simulink model "s_c107m32k_vlbi"  (R2018a)
settings: Solver=VariableStepDiscrete  StartTime=0.0  StopTime=(2^15)*10  RelTol=1e-3
undefined symbols (not defined in the file): fft_stages, n_bits_xengs
libraries: xbsIndex_r4 x23049, casper_library_misc x45, xps_library x4, casper_library_scopes x3, simulink x2
(part 5 of 201)

== system s_c107m32k_vlbi/DDC ==
  note: Sync and DV will be inline here
  note: DDS 18.17
  note: Mixer
  note: Filter
  note: Developers note: The coeffs are baked into the block 'UserData' area.
      | The Coeffs are supplied by System Engineering, except implmented at better
      | precision (previous commits the precision was rounded up to 6 decimal places).
      | The coeffs have been added to the User_Data area in the ddc_fir_async
      | blocks (set_param(gcb, 'UserData', coef_107M_6dB_equiripple2) where
      | coef_107M_6dB_equiripple2 was supplied in a .mat file from SE.
      | The coeffs should now 'travel' with the model in full precision.
      | To access: getfield(get_param(gcb, 'UserData'), 'parameters','coeff')
      | is used in the top level model mask.
  sync : Inport
  dvalid : Inport  Port=2
  pol0_data : Inport  Port=3
  osc0 : Inport  Port=4
  pol1_data : Inport  Port=5
  osc1 : Inport  Port=6
  Assert : xbsIndex_r4/Assert  assert_type=on  type_source=Explicitly  gui_display_data_type=Boolean  arith_type=Boolean  n_bits=16  bin_pt=14  preci_type=Single  exp_width=8  frac_width=24  assert_rate=off  rate_source=Explicitly  period=1  output_port=on  block_type=assert
  Concat : xbsIndex_r4/Concat  num_inputs=2  dbl_ovrd=off  block_type=concat
  Concat1 : xbsIndex_r4/Concat  num_inputs=2  dbl_ovrd=off  block_type=concat
  Concat2 : xbsIndex_r4/Concat  num_inputs=2  dbl_ovrd=off  block_type=concat
  Constant : xbsIndex_r4/Constant  const=0  gui_display_data_type=Fixed-point  arith_type=Unsigned  n_bits=8  bin_pt=0  preci_type=Single  exp_width=8  frac_width=24  explicit_period=on  period=1  equ=P=C  opselect=C  inp2=PCIN>>17  opr=+  inp1=P  carry=CIN  dbl_ovrd=off  block_type=constant
  Counter1 : xbsIndex_r4/Counter  Commented=on  cnt_type=Free Running  cnt_to=Inf  operation=Up  start_count=0  cnt_by_val=1  arith_type=Unsigned  n_bits=8  bin_pt=0  load_pin=off  rst=on  en=on  explicit_period=on  period=1  use_behavioral_HDL=off  implementation=DSP48  dbl_ovrd=off  block_type=counter
      settings: block_version=11.4
  Counter2 : xbsIndex_r4/Counter  Commented=on  cnt_type=Free Running  cnt_to=Inf  operation=Up  start_count=0  cnt_by_val=1  arith_type=Unsigned  n_bits=32  bin_pt=0  load_pin=off  rst=on  en=on  explicit_period=on  period=1  use_behavioral_HDL=off  implementation=Fabric  dbl_ovrd=off  block_type=counter
  Counter3 : xbsIndex_r4/Counter  Commented=on  cnt_type=Free Running  cnt_to=Inf  operation=Up  start_count=0  cnt_by_val=1  arith_type=Unsigned  n_bits=8  bin_pt=0  load_pin=off  rst=on  en=on  explicit_period=on  period=1  use_behavioral_HDL=off  implementation=DSP48  dbl_ovrd=off  block_type=counter
      settings: block_version=11.4
  Counter33 : xbsIndex_r4/Counter  Commented=on  cnt_type=Free Running  cnt_to=Inf  operation=Up  start_count=0  cnt_by_val=1  arith_type=Unsigned  n_bits=32  bin_pt=0  load_pin=off  rst=on  en=on  explicit_period=on  period=1  use_behavioral_HDL=off  implementation=Fabric  dbl_ovrd=off  block_type=counter
  Counter4 : xbsIndex_r4/Counter  Commented=on  cnt_type=Free Running  cnt_to=Inf  operation=Up  start_count=0  cnt_by_val=1  arith_type=Unsigned  n_bits=32  bin_pt=0  load_pin=off  rst=on  en=off  explicit_period=on  period=1  use_behavioral_HDL=off  implementation=Fabric  dbl_ovrd=off  block_type=counter
  Counter46 : xbsIndex_r4/Counter  Commented=on  cnt_type=Free Running  cnt_to=Inf  operation=Up  start_count=0  cnt_by_val=1  arith_type=Unsigned  n_bits=32  bin_pt=0  load_pin=off  rst=on  en=off  explicit_period=on  period=1  use_behavioral_HDL=off  implementation=Fabric  dbl_ovrd=off  block_type=counter
  Delay{1..2,4,6..9} (7 alike) : xbsIndex_r4/Delay  rst=off  infoeditControl=Selection of Reset will increase slice count due to use of real FFs and instead of SRLs  en=off  latency=1  reg_retiming=off  dbl_ovrd=off  block_type=delay
      settings: infoedit=Hardware notes: A delay line is a chain, each link of which is an SRL16 or SRL32 followed by a flip-flop.
  Delay3 : xbsIndex_r4/Delay  rst=off  infoeditControl=Selection of Reset will increase slice count due to use of real FFs and instead of SRLs  en=on  latency=1  reg_retiming=off  dbl_ovrd=off  block_type=delay
      settings: infoedit=Hardware notes: A delay line is a chain, each link of which is an SRL16 or SRL32 followed by a flip-flop.
  Delay5 : xbsIndex_r4/Delay  rst=off  infoeditControl=Selection of Reset will increase slice count due to use of real FFs and instead of SRLs  en=on  latency=1  reg_retiming=off  dbl_ovrd=off  block_type=delay
      settings: infoedit=Hardware notes: A delay line is a chain, each link of which is an SRL16 or SRL32 followed by a flip-flop.
  From{2,6,13,16,18,21,33} (7 alike) : From  Commented=on  GotoTag=dec_sync  TagVisibility=global
  From{4,17,22,34} (4 alike) : From  Commented=on  GotoTag=ddc_sync
  From19 : From  Commented=on  GotoTag=dec_d80_0  TagVisibility=global
  From20 : From  Commented=on  GotoTag=cnt_rst  TagVisibility=global
      settings: CloseFcn=tagdialog Close
  From23 : From  Commented=on  GotoTag=ddc_pol0
  From28 : From  Commented=on  GotoTag=cnt_rst  TagVisibility=global
      settings: CloseFcn=tagdialog Close
  From3 : From  Commented=on  GotoTag=dec_dv  TagVisibility=global
  Gateway Out1 : xbsIndex_r4/Gateway Out  inherit_from_input=off  hdl_port=on  rows=1  columns=1  UseAsDAC=off  DACChannel='1'  interface=None  automatic_assignment=on  address_offset=hex2dec('00')  intf_name=''  intf_description=''  timing_constraint=None  locs_specified=off  LOCs={}  io_standard={}  block_type=gatewayout
  Gateway Out2 : xbsIndex_r4/Gateway Out  inherit_from_input=off  hdl_port=on  rows=1  columns=1  UseAsDAC=off  DACChannel='1'  interface=None  automatic_assignment=on  address_offset=hex2dec('00')  intf_name=''  intf_description=''  timing_constraint=None  locs_specified=off  LOCs={}  io_standard={}  block_type=gatewayout
  Inverter : xbsIndex_r4/Inverter  en=off  latency=0  dbl_ovrd=off  block_type=inv
  Logical : xbsIndex_r4/Logical  Commented=on  logical_function=OR  inputs=2  en=off  latency=0  precision=Full  arith_type=Unsigned  n_bits=16  bin_pt=0  align_bp=on  dbl_ovrd=off  block_type=logical
  Logical1 : xbsIndex_r4/Logical  logical_function=AND  inputs=2  en=off  latency=0  precision=Full  arith_type=Unsigned  n_bits=16  bin_pt=0  align_bp=on  dbl_ovrd=off  block_type=logical
  Logical2 : xbsIndex_r4/Logical  logical_function=AND  inputs=2  en=off  latency=0  precision=Full  arith_type=Unsigned  n_bits=16  bin_pt=0  align_bp=on  dbl_ovrd=off  block_type=logical
  Logical29 : xbsIndex_r4/Logical  Commented=on  logical_function=AND  inputs=2  en=off  latency=0  precision=Full  arith_type=Unsigned  n_bits=16  bin_pt=0  align_bp=on  dbl_ovrd=off  block_type=logical
  Logical3 : xbsIndex_r4/Logical  Commented=on  logical_function=AND  inputs=2  en=off  latency=0  precision=Full  arith_type=Unsigned  n_bits=16  bin_pt=0  align_bp=on  dbl_ovrd=off  block_type=logical
  Register : xbsIndex_r4/Register  init=0  rst=off  en=on  dbl_ovrd=off  block_type=register
  Register1 : xbsIndex_r4/Register  init=0  rst=on  en=on  dbl_ovrd=off  block_type=register
  Register2 : xbsIndex_r4/Register  init=0  rst=on  en=on  dbl_ovrd=off  block_type=register
  Register{4..7,24,37,49,62} (8 alike) : xbsIndex_r4/Register  Commented=on  init=0  rst=on  en=on  dbl_ovrd=off  block_type=register
  Register3 : xbsIndex_r4/Register  init=0  rst=off  en=on  dbl_ovrd=off  block_type=register
  Relational : xbsIndex_r4/Relational  mode=a!=b  op_type=Bool  en=off  latency=1  dbl_ovrd=off  block_type=relational
  Relational1 : xbsIndex_r4/Relational  mode=a!=b  op_type=Bool  en=off  latency=1  dbl_ovrd=off  block_type=relational
  Slice1 : xbsIndex_r4/Slice  Commented=on  nbits=32  boolean_output=off  mode=Lower Bit Location + Width  bit1=0  base1=MSB of Input  bit0=0  base0=LSB of Input  dbl_ovrd=off  block_type=slice
  Slice34 : xbsIndex_r4/Slice  Commented=on  nbits=32  boolean_output=off  mode=Lower Bit Location + Width  bit1=0  base1=MSB of Input  bit0=0  base0=LSB of Input  dbl_ovrd=off  block_type=slice
  Terminator : Terminator
  Terminator1 : Terminator
  To Workspace1 : ToWorkspace  VariableName=mult_sync  SaveFormat=Timeseries  SampleTime=-1
  To Workspace2 : ToWorkspace  VariableName=mult_dv  SaveFormat=Timeseries  SampleTime=-1
  bus_convert : Subsystem  AncestorBlock=casper_library_bus/bus_convert  mask(bus_convert){n_bits_in=[29 29 29 29 29 29 29 29], bin_pt_in=26, cmplx=on, n_bits_out=18, bin_pt_out=17, quantization=2, overflow=1, csp_latency=2, of=on, misc=on}
      mask prompts: n_bits_in "input bit widths"; bin_pt_in "input binary points"; cmplx "input complex"; n_bits_out "output bit widths"; bin_pt_out "output binary points"; quantization "quantization strategy (Truncate=0, Round  (unbiased: +/- Inf)=1, Round (unbiased: Even Values)=2)"; overflow "overflow strategy (Wrap=0, Saturate=1, Flag as error=2)"; csp_latency "latency"; of "overflow indication"; misc "misc support"
      mask help: Convert components of busses
      mask init:
      | bus_convert_init(gcb, ...
      |     'n_bits_in', n_bits_in, ...
      |     'bin_pt_in', bin_pt_in, ...
      |     'cmplx', cmplx, ...
      |     'n_bits_out', n_bits_out, ...
      |     'bin_pt_out', bin_pt_out, ...
      |     'quantization', quantization, ...
      |     'overflow', overflow, ...
      |     'csp_latency', csp_latency, ...
      |     'misc', misc, ...
      |     'of', of);
  bus_convert1 : Subsystem  AncestorBlock=casper_library_bus/bus_convert  mask(bus_convert){n_bits_in=[29 29 29 29 29 29 29 29], bin_pt_in=26, cmplx=on, n_bits_out=18, bin_pt_out=17, quantization=2, overflow=1, csp_latency=2, of=on, misc=off}
      mask prompts: n_bits_in "input bit widths"; bin_pt_in "input binary points"; cmplx "input complex"; n_bits_out "output bit widths"; bin_pt_out "output binary points"; quantization "quantization strategy (Truncate=0, Round  (unbiased: +/- Inf)=1, Round (unbiased: Even Values)=2)"; overflow "overflow strategy (Wrap=0, Saturate=1, Flag as error=2)"; csp_latency "latency"; of "overflow indication"; misc "misc support"
      mask help: Convert components of busses
      mask init: same as s_c107m32k_vlbi/DDC/bus_convert
  bus_expand : Subsystem  mask(bus_expand){mode=divisions of equal size, outputNum=2, outputWidth=1, outputBinaryPt=0, outputArithmeticType=2, show_format=off, outputToWorkspace=off, variablePrefix=out, outputToModelAsWell=on}
      mask prompts: outputNum "Number of outputs:"; outputWidth "Output width:"; outputBinaryPt "Output binary point position:"; outputArithmeticType "Output arithmetic type (ufix=0, fix=1, bool=2):"; show_format "Print format string?"; outputToWorkspace "Output to workspace?"; variablePrefix "Variable name prefix:"; outputToModelAsWell "Output to model as well?"
      mask help:
      | Expands a 'bus' made using a bus_create or Xilinx
      | concat block.
      | The input will be divided into the specified number
      | of outputs with the specified arithmetic types.
      | Divisions are made from most significant bit.
      mask init: same as s_c107m32k_vlbi/bus_expand1
      settings: AttributesFormatString=2 outputs
      mask TypeOptions mode: divisions of equal size | divisions of arbitrary size
      mask Callback mode: bus_expand_callback();
      mask Callback outputWidth: bus_expand_callback();
      mask Callback outputToWorkspace: bus_expand_callback();
  bus_expand1 : Subsystem  mask(bus_expand){mode=divisions of equal size, outputNum=16, outputWidth=18, outputBinaryPt=17, outputArithmeticType=1, show_format=off, outputToWorkspace=off, variablePrefix=Sin, outputToModelAsWell=off}
      mask prompts: outputNum "Number of outputs:"; outputWidth "Output width:"; outputBinaryPt "Output binary point position:"; outputArithmeticType "Output arithmetic type (ufix=0, fix=1, bool=2):"; show_format "Print format string?"; outputToWorkspace "Output to workspace?"; variablePrefix "Variable name prefix:"; outputToModelAsWell "Output to model as well?"
      mask help:
      | Expands a 'bus' made using a bus_create or Xilinx
      | concat block.
      | The input will be divided into the specified number
      | of outputs with the specified arithmetic types.
      | Divisions are made from most significant bit.
      mask init: same as s_c107m32k_vlbi/bus_expand1
      settings: AttributesFormatString=16 outputs
      mask TypeOptions mode: divisions of equal size | divisions of arbitrary size
      mask Callback mode: bus_expand_callback();
      mask Callback outputWidth: bus_expand_callback();
      mask Callback outputToWorkspace: bus_expand_callback();
  bus_expand2 : Subsystem  mask(bus_expand){mode=divisions of equal size, outputNum=16, outputWidth=18, outputBinaryPt=17, outputArithmeticType=1, show_format=off, outputToWorkspace=off, variablePrefix=Sin, outputToModelAsWell=off}
      mask prompts: outputNum "Number of outputs:"; outputWidth "Output width:"; outputBinaryPt "Output binary point position:"; outputArithmeticType "Output arithmetic type (ufix=0, fix=1, bool=2):"; show_format "Print format string?"; outputToWorkspace "Output to workspace?"; variablePrefix "Variable name prefix:"; outputToModelAsWell "Output to model as well?"
      mask help:
      | Expands a 'bus' made using a bus_create or Xilinx
      | concat block.
      | The input will be divided into the specified number
      | of outputs with the specified arithmetic types.
      | Divisions are made from most significant bit.
      mask init: same as s_c107m32k_vlbi/bus_expand1
      settings: AttributesFormatString=16 outputs
      mask TypeOptions mode: divisions of equal size | divisions of arbitrary size
      mask Callback mode: bus_expand_callback();
      mask Callback outputWidth: bus_expand_callback();
      mask Callback outputToWorkspace: bus_expand_callback();
  bus_expand5 : Subsystem  mask(bus_expand){mode=divisions of equal size, outputNum=16, outputWidth=18, outputBinaryPt=17, outputArithmeticType=1, show_format=off, outputToWorkspace=off, variablePrefix=Sin, outputToModelAsWell=off}
      mask prompts: outputNum "Number of outputs:"; outputWidth "Output width:"; outputBinaryPt "Output binary point position:"; outputArithmeticType "Output arithmetic type (ufix=0, fix=1, bool=2):"; show_format "Print format string?"; outputToWorkspace "Output to workspace?"; variablePrefix "Variable name prefix:"; outputToModelAsWell "Output to model as well?"
      mask help:
      | Expands a 'bus' made using a bus_create or Xilinx
      | concat block.
      | The input will be divided into the specified number
      | of outputs with the specified arithmetic types.
      | Divisions are made from most significant bit.
      mask init: same as s_c107m32k_vlbi/bus_expand1
      settings: AttributesFormatString=16 outputs
      mask TypeOptions mode: divisions of equal size | divisions of arbitrary size
      mask Callback mode: bus_expand_callback();
      mask Callback outputWidth: bus_expand_callback();
      mask Callback outputToWorkspace: bus_expand_callback();
  bus_expand6 : Subsystem  mask(bus_expand){mode=divisions of equal size, outputNum=16, outputWidth=18, outputBinaryPt=17, outputArithmeticType=1, show_format=off, outputToWorkspace=off, variablePrefix=Sin, outputToModelAsWell=off}
      mask prompts: outputNum "Number of outputs:"; outputWidth "Output width:"; outputBinaryPt "Output binary point position:"; outputArithmeticType "Output arithmetic type (ufix=0, fix=1, bool=2):"; show_format "Print format string?"; outputToWorkspace "Output to workspace?"; variablePrefix "Variable name prefix:"; outputToModelAsWell "Output to model as well?"
      mask help:
      | Expands a 'bus' made using a bus_create or Xilinx
      | concat block.
      | The input will be divided into the specified number
      | of outputs with the specified arithmetic types.
      | Divisions are made from most significant bit.
      mask init: same as s_c107m32k_vlbi/bus_expand1
      settings: AttributesFormatString=16 outputs
      mask TypeOptions mode: divisions of equal size | divisions of arbitrary size
      mask Callback mode: bus_expand_callback();
      mask Callback outputWidth: bus_expand_callback();
      mask Callback outputToWorkspace: bus_expand_callback();
  bus_mult : Subsystem  mask(bus_mult){n_bits_a=[10,10,10,10,10,10,10,10], bin_pt_a=9, type_a=1, cmplx_a=on, n_bits_b=[18,18,18,18,18,18,18,18], bin_pt_b=17, type_b=1, cmplx_b=on, misc=on, floating_point=off, float_type=single, input_vec_a=1, input_vec_b=1, frac_width=19, exp_width=6, n_bits_out=29, bin_pt_out=26, type_out=1, quantization=0, overflow=0, mult_latency=7, add_latency=7, conv_latency=0, max_fanout=1, fan_latency=1, multiplier_implementation=embedded multiplier core, pipeline_cmult_en=off, pipeline_latency=0}
      mask prompts: n_bits_a "a input bit widths"; bin_pt_a "a input binary points"; type_a "a input type (Unsigned=0, Signed=1)"; cmplx_a "a input complex"; n_bits_b "b input bit widths"; bin_pt_b "b input binary points"; type_b "b input type (Unsigned=0, Signed=1)"; cmplx_b "b input complex"; misc "misc support"; floating_point "floating point"; float_type "float type"; input_vec_a "a input vector in bus"; input_vec_b "b input vector in bus"; frac_width "fraction width"; exp_width "exponent width"; n_bits_out "output bit widths"; bin_pt_out "output binary points"; type_out "output type (Unsigned=0, Signed=1)"; quantization "quantization strategy (Truncate=0, Round  (unbiased: +/- Inf)=1)"; overflow "overflow strategy (Wrap=0, Saturate=1, Flag as error=2)"; mult_latency "multiplier latency"; add_latency "adder latency"; conv_latency "convert latency"; max_fanout "limit fanout to ?"; fan_latency "fanout register latency"; multiplier_implementation "multiplier implementation"; pipeline_cmult_en "pipeline complex mult"; pipeline_latency "pipeline latency"
      mask help: Multiply components of two busses
      mask init:
      | bus_mult_init(gcb, ...
      |     'n_bits_a', n_bits_a, ...
      |     'bin_pt_a', bin_pt_a, ...
      |     'type_a', type_a, ...
      |     'cmplx_a', cmplx_a, ...
      |     'n_bits_b', n_bits_b, ...
      |     'bin_pt_b', bin_pt_b, ...
      |     'type_b', type_b, ...
      |     'cmplx_b', cmplx_b, ...
      |     'n_bits_out', n_bits_out, ...
      |     'bin_pt_out', bin_pt_out, ...
      |     'type_out', type_out, ...
      |     'floating_point', floating_point, ...
      |     'float_type', float_type, ...
      |     'exp_width', exp_width, ...
      |     'input_vec_a', input_vec_a, ...
      |     'input_vec_b', input_vec_b, ...
      |     'frac_width', frac_width, ...         
      |     'quantization', quantization, ...
      |     'overflow', overflow, ...
      |     'mult_latency', mult_latency, ...
      |     'add_latency', add_latency, ...
      |     'conv_latency', conv_latency, ...
      |     'max_fanout', max_fanout, ...
      |     'pipeline_cmult_en', pipeline_cmult_en, ...
      |     'pipeline_latency', pipeline_latency, ...
      |     'fan_latency', fan_latency, ...
      |     'multiplier_implementation', multiplier_implementation, ...
      |     'misc', misc);
      mask Callback floating_point:
      | onoff = get_param(gcb, 'floating_point');
      | if strcmp(onoff,'on')
      |     enable_fixpt = 'off'
      |     set_param_state(gcb, 'float_type', 'on')
      | 
      |     set_param_state(gcb, 'input_vec_a', 'on')
      |     set_param_state(gcb, 'input_vec_b', 'on')
      | 
      |     f_type = get_param(gcb, 'float_type')
      |     if strcmp(f_type,'custom')
      |         set_param_state(gcb, 'exp_width', 'on')
      |         set_param_state(gcb, 'frac_width', 'on')
      |     else
      |         set_param_state(gcb, 'exp_width', 'off')
      |         set_param_state(gcb, 'frac_width', 'off')
      |     end
      | 
      | else
      |     enable_fixpt = 'on'
      |     set_param_state(gcb, 'float_type', 'off')
      |     set_param_state(gcb, 'exp_width', 'off')
      |     set_param_state(gcb, 'frac_width', 'off')
      |     set_param_state(gcb, 'input_vec_a', 'off')
      |     set_param_state(gcb, 'input_vec_b', 'off')
      | end
      | 
      | set_param_state(gcb, 'n_bits_a', enable_fixpt)
      | set_param_state(gcb, 'bin_pt_a', enable_fixpt)
      | set_param_state(gcb, 'type_a', enable_fixpt)
      | set_param_state(gcb, 'n_bits_b', enable_fixpt)
      | set_param_state(gcb, 'bin_pt_b', enable_fixpt)
      | set_param_state(gcb, 'type_b', enable_fixpt)
      | 
      | set_param_state(gcb, 'n_bits_out', enable_fixpt)
      | set_param_state(gcb, 'bin_pt_out', enable_fixpt)
      | set_param_state(gcb, 'type_out', enable_fixpt)
      | set_param_state(gcb, 'quantization', enable_fixpt)
      | set_param_state(gcb, 'overflow', enable_fixpt)
      mask TypeOptions float_type: single | custom
      mask Callback float_type:
      | f_type = get_param(gcb, 'float_type')
      | if strcmp(f_type,'custom')
      |     set_param_state(gcb, 'exp_width', 'on')
      |     set_param_state(gcb, 'frac_width', 'on')
      | else
      |     set_param_state(gcb, 'exp_width', 'off')
      |     set_param_state(gcb, 'frac_width', 'off')
      | end
      mask TypeOptions multiplier_implementation: behavioral HDL | standard core | embedded multiplier core
      mask Callback pipeline_cmult_en:
      | pipeline_en = get_param(gcb, 'pipeline_cmult_en');
      | if strcmp(pipeline_en,'on')
      | 
      |     set_param_state(gcb, 'pipeline_latency', 'on')
      | else
      |     set_param_state(gcb, 'pipeline_latency', 'off')
      | end
  bus_mult1 : Subsystem  mask(bus_mult){n_bits_a=[10,10,10,10,10,10,10,10], bin_pt_a=9, type_a=1, cmplx_a=on, n_bits_b=[18,18,18,18,18,18,18,18], bin_pt_b=17, type_b=1, cmplx_b=on, misc=off, floating_point=off, float_type=single, input_vec_a=1, input_vec_b=1, frac_width=19, exp_width=6, n_bits_out=29, bin_pt_out=26, type_out=1, quantization=0, overflow=0, mult_latency=7, add_latency=7, conv_latency=0, max_fanout=1, fan_latency=1, multiplier_implementation=embedded multiplier core, pipeline_cmult_en=off, pipeline_latency=0}
      mask prompts: n_bits_a "a input bit widths"; bin_pt_a "a input binary points"; type_a "a input type (Unsigned=0, Signed=1)"; cmplx_a "a input complex"; n_bits_b "b input bit widths"; bin_pt_b "b input binary points"; type_b "b input type (Unsigned=0, Signed=1)"; cmplx_b "b input complex"; misc "misc support"; floating_point "floating point"; float_type "float type"; input_vec_a "a input vector in bus"; input_vec_b "b input vector in bus"; frac_width "fraction width"; exp_width "exponent width"; n_bits_out "output bit widths"; bin_pt_out "output binary points"; type_out "output type (Unsigned=0, Signed=1)"; quantization "quantization strategy (Truncate=0, Round  (unbiased: +/- Inf)=1)"; overflow "overflow strategy (Wrap=0, Saturate=1, Flag as error=2)"; mult_latency "multiplier latency"; add_latency "adder latency"; conv_latency "convert latency"; max_fanout "limit fanout to ?"; fan_latency "fanout register latency"; multiplier_implementation "multiplier implementation"; pipeline_cmult_en "pipeline complex mult"; pipeline_latency "pipeline latency"
      mask help: Multiply components of two busses
      mask init: same as s_c107m32k_vlbi/DDC/bus_mult
      mask Callback floating_point:
      | onoff = get_param(gcb, 'floating_point');
      | if strcmp(onoff,'on')
      |     enable_fixpt = 'off'
      |     set_param_state(gcb, 'float_type', 'on')
      | 
      |     set_param_state(gcb, 'input_vec_a', 'on')
      |     set_param_state(gcb, 'input_vec_b', 'on')
      | 
      |     f_type = get_param(gcb, 'float_type')
      |     if strcmp(f_type,'custom')
      |         set_param_state(gcb, 'exp_width', 'on')
      |         set_param_state(gcb, 'frac_width', 'on')
      |     else
      |         set_param_state(gcb, 'exp_width', 'off')
      |         set_param_state(gcb, 'frac_width', 'off')
      |     end
      | 
      | else
      |     enable_fixpt = 'on'
      |     set_param_state(gcb, 'float_type', 'off')
      |     set_param_state(gcb, 'exp_width', 'off')
      |     set_param_state(gcb, 'frac_width', 'off')
      |     set_param_state(gcb, 'input_vec_a', 'off')
      |     set_param_state(gcb, 'input_vec_b', 'off')
      | end
      | 
      | set_param_state(gcb, 'n_bits_a', enable_fixpt)
      | set_param_state(gcb, 'bin_pt_a', enable_fixpt)
      | set_param_state(gcb, 'type_a', enable_fixpt)
      | set_param_state(gcb, 'n_bits_b', enable_fixpt)
      | set_param_state(gcb, 'bin_pt_b', enable_fixpt)
      | set_param_state(gcb, 'type_b', enable_fixpt)
      | 
      | set_param_state(gcb, 'n_bits_out', enable_fixpt)
      | set_param_state(gcb, 'bin_pt_out', enable_fixpt)
      | set_param_state(gcb, 'type_out', enable_fixpt)
      | set_param_state(gcb, 'quantization', enable_fixpt)
      | set_param_state(gcb, 'overflow', enable_fixpt)
      mask TypeOptions float_type: single | custom
      mask Callback float_type:
      | f_type = get_param(gcb, 'float_type')
      | if strcmp(f_type,'custom')
      |     set_param_state(gcb, 'exp_width', 'on')
      |     set_param_state(gcb, 'frac_width', 'on')
      | else
      |     set_param_state(gcb, 'exp_width', 'off')
      |     set_param_state(gcb, 'frac_width', 'off')
      | end
      mask TypeOptions multiplier_implementation: behavioral HDL | standard core | embedded multiplier core
      mask Callback pipeline_cmult_en:
      | pipeline_en = get_param(gcb, 'pipeline_cmult_en');
      | if strcmp(pipeline_en,'on')
      | 
      |     set_param_state(gcb, 'pipeline_latency', 'on')
      | else
      |     set_param_state(gcb, 'pipeline_latency', 'off')
      | end
  convert_of : Subsystem  Commented=on  AncestorBlock=casper_library_misc/convert_of  mask(convert_of){bit_width_i=44, binary_point_i=34, bit_width_o=18, binary_point_o=17, latency=2, overflow=Saturate, quantization=Round  (unbiased: +/- Inf)}
      mask prompts: bit_width_i "Bit Width In"; binary_point_i "Binary Point In"; bit_width_o "Bit Width Out"; binary_point_o "Binary Point Out"; overflow "Overflow Behaviour"; quantization "Quantization Behaviour"
      mask help:
      | Converts from one 2's complement bit-width
      | and/or binary point position to another.
      | Includes underflow/overflow indicator.
      mask init:
      | convert_of_init(gcb, ...
      |     'bit_width_i', bit_width_i, ...
      |     'binary_point_i', binary_point_i, ...
      |     'bit_width_o', bit_width_o, ...
      |     'binary_point_o', binary_point_o, ...
      |     'latency', latency, ...
      |     'overflow', overflow, ...
      |     'quantization', quantization);
      settings: AttributesFormatString=[44,34]->[18,17]
      mask TypeOptions overflow: Wrap | Saturate | Error
      mask TypeOptions quantization: Truncate | Round  (unbiased: +/- Inf) | Round  (unbiased: even values)
  convert_of1 : Subsystem  Commented=on  AncestorBlock=casper_library_misc/convert_of  mask(convert_of){bit_width_i=44, binary_point_i=34, bit_width_o=18, binary_point_o=17, latency=2, overflow=Saturate, quantization=Round  (unbiased: +/- Inf)}
      mask prompts: bit_width_i "Bit Width In"; binary_point_i "Binary Point In"; bit_width_o "Bit Width Out"; binary_point_o "Binary Point Out"; overflow "Overflow Behaviour"; quantization "Quantization Behaviour"
      mask help:
      | Converts from one 2's complement bit-width
      | and/or binary point position to another.
      | Includes underflow/overflow indicator.
      mask init: same as s_c107m32k_vlbi/DDC/convert_of
      settings: AttributesFormatString=[44,34]->[18,17]
      mask TypeOptions overflow: Wrap | Saturate | Error
      mask TypeOptions quantization: Truncate | Round  (unbiased: +/- Inf) | Round  (unbiased: even values)
  ddc_in_sync_cnt : Subsystem  Tag=xps:sw_reg  Commented=on  AncestorBlock=xps_library/Memory/software_register  mask(swreg){io_dir=To Processor, io_delay=0, init_val=0, sample_period=1, names=reg, bitwidths=8, bin_pts=0, arith_types=0, sim_port=off, show_format=on}
      mask prompts: io_dir "I/O direction"; io_delay "I/O delay"; init_val "Initial Value"; sample_period "Sample period"; names "Bitfield names [msb...lsb]"; bitwidths "Bitfield widths"; bin_pts "Bitfield binary pts"; arith_types "Bitfield types, ufix=0, fix=1, bool=2"; sim_port "Provide sim input/output?"; show_format "Print format string?"
      mask help: A 32-bit software-accessible register. Can be divided into bitfields of varying widths and types using the fields in the block mask.
      mask init:
      | swreg_init(gcb)
      settings: AttributesFormatString=1output:uf8.0 = 8 bits
      mask TypeOptions io_dir: To Processor | From Processor
      mask Callback io_dir:
      | mask_enables = get_param(gcb, 'MaskEnables');
      | mask_names = get_param(gcb, 'MaskNames');
      | if strcmp(get_param(gcb, 'io_dir'), 'To Processor'),
      |     mask_enables{ismember(mask_names, 'sample_period')} = 'off';
      | else
      |     mask_enables{ismember(mask_names, 'sample_period')} = 'on';
      | end
      | set_param(gcb, 'MaskEnables', mask_enables);
      mask DialogControl ParameterTabVar0 Prompt: Setup
  ddc_out_sync_cnt : Subsystem  Tag=xps:sw_reg  Commented=on  AncestorBlock=xps_library/Memory/software_register  mask(swreg){io_dir=To Processor, io_delay=0, init_val=0, sample_period=1, names=reg, bitwidths=8, bin_pts=0, arith_types=0, sim_port=off, show_format=on}
      mask prompts: io_dir "I/O direction"; io_delay "I/O delay"; init_val "Initial Value"; sample_period "Sample period"; names "Bitfield names [msb...lsb]"; bitwidths "Bitfield widths"; bin_pts "Bitfield binary pts"; arith_types "Bitfield types, ufix=0, fix=1, bool=2"; sim_port "Provide sim input/output?"; show_format "Print format string?"
      mask help: A 32-bit software-accessible register. Can be divided into bitfields of varying widths and types using the fields in the block mask.
      mask init:
      | swreg_init(gcb)
      settings: AttributesFormatString=1output:uf8.0 = 8 bits
      mask TypeOptions io_dir: To Processor | From Processor
      mask Callback io_dir:
      | mask_enables = get_param(gcb, 'MaskEnables');
      | mask_names = get_param(gcb, 'MaskNames');
      | if strcmp(get_param(gcb, 'io_dir'), 'To Processor'),
      |     mask_enables{ismember(mask_names, 'sample_period')} = 'off';
      | else
      |     mask_enables{ismember(mask_names, 'sample_period')} = 'on';
      | end
      | set_param(gcb, 'MaskEnables', mask_enables);
      mask DialogControl ParameterTabVar0 Prompt: Setup
  dec_fir_async : Subsystem  Tag=casper:dec_fir_async  AncestorBlock=casper_library_downconverter/dec_fir_async  mask(dec_fir_async){n_inputs=16, coeff=getfield(get_param(gcb, 'UserData'), 'parameters','coeff'), output_width=18, output_bp=17, quantization=Round  (unbiased: Even Values), add_latency=7, mult_latency=7, conv_latency=7, coeff_bit_width=18, coeff_bin_pt=17, lshift=0, absorb_adders=on, adder_imp=DSP48, async=on, bus_input=off, input_width=0, input_bp=0, input_type=Signed}
      mask prompts: n_inputs "Number of Parallel Streams"; coeff "Coefficients"; output_width "Output bitwidth"; output_bp "Output binary point"; quantization "Quantization Behavior"; add_latency "Add Latency"; mult_latency "Mult Latency"; conv_latency "Convert latency"; coeff_bit_width "Coefficient bitwidth"; coeff_bin_pt "Coefficient binary point"; lshift "Post adder-tree shift"; absorb_adders "Absorb adders into DSP slices"; adder_imp "Adder implementation"; async "Asynchronous ops"; bus_input "Bus input"; input_width "Input bitwidth"; input_bp "Input binary point"; input_type "Input datatype"
      mask help: FIR filter which can handle multiple time samples in parallel and decimates down to 1 time sample. If coefficients are symmetric, will automatically fold before multiplying.
      mask init:
      | dec_fir_async_init(gcb);
      settings: AttributesFormatString=|
      | 256 taps
      | 18_17 r/i
      mask TypeOptions quantization: Truncate | Round  (unbiased: +/- Inf) | Round  (unbiased: Even Values)
      mask TypeOptions adder_imp: Behavioral | Fabric | DSP48
      mask Callback bus_input:
      | onoff = get_param(gcb, 'bus_input');
      | set_param_state(gcb, 'input_width', onoff)
      | set_param_state(gcb, 'input_bp', onoff)
      | set_param_state(gcb, 'input_type', onoff)
      mask TypeOptions input_type: Signed | Unsigned
  dec_fir_async2 : Subsystem  Tag=casper:dec_fir_async  AncestorBlock=casper_library_downconverter/dec_fir_async  mask(dec_fir_async){n_inputs=16, coeff=getfield(get_param(gcb, 'UserData'), 'parameters','coeff'), output_width=18, output_bp=17, quantization=Round  (unbiased: Even Values), add_latency=7, mult_latency=7, conv_latency=7, coeff_bit_width=18, coeff_bin_pt=17, lshift=0, absorb_adders=on, adder_imp=DSP48, async=on, bus_input=off, input_width=0, input_bp=0, input_type=Signed}
      mask prompts: n_inputs "Number of Parallel Streams"; coeff "Coefficients"; output_width "Output bitwidth"; output_bp "Output binary point"; quantization "Quantization Behavior"; add_latency "Add Latency"; mult_latency "Mult Latency"; conv_latency "Convert latency"; coeff_bit_width "Coefficient bitwidth"; coeff_bin_pt "Coefficient binary point"; lshift "Post adder-tree shift"; absorb_adders "Absorb adders into DSP slices"; adder_imp "Adder implementation"; async "Asynchronous ops"; bus_input "Bus input"; input_width "Input bitwidth"; input_bp "Input binary point"; input_type "Input datatype"
      mask help: FIR filter which can handle multiple time samples in parallel and decimates down to 1 time sample. If coefficients are symmetric, will automatically fold before multiplying.
      mask init:
      | dec_fir_async_init(gcb);
      settings: AttributesFormatString=|
      | 256 taps
      | 18_17 r/i
      mask TypeOptions quantization: Truncate | Round  (unbiased: +/- Inf) | Round  (unbiased: Even Values)
      mask TypeOptions adder_imp: Behavioral | Fabric | DSP48
      mask Callback bus_input:
      | onoff = get_param(gcb, 'bus_input');
      | set_param_state(gcb, 'input_width', onoff)
      | set_param_state(gcb, 'input_bp', onoff)
      | set_param_state(gcb, 'input_type', onoff)
      mask TypeOptions input_type: Signed | Unsigned
  edge_detect1 : Subsystem  Commented=on  mask(edge_detect){edge=Rising, polarity=Active High, x_in=[0 0.08 0.08 0.16 0.16 0.24 0.24 0.32 0.32 0.4], y_in=[-1 -1  1  1  1  1  1  1  1  1], x_out=[0.6 0.68 0.68 0.76 0.76 0.84 0.84 0.92 0.92 1], y_out=[-1 -1  1  1 -1 -1 -1 -1 -1 -1]}
      mask prompts: edge "Edge Type"; polarity "Output Polarity"; x_in "Input X Positions"; y_in "Input Y Positions"; x_out "Output X Positions"; y_out "Output Y Positions"
      mask help: Output is active for one-cycle after each edge of the specified type (i.e. rising, falling or both).
      mask init: same as s_c107m32k_vlbi/edge_detect1
      settings: AttributesFormatString=|
      | rising edges
      | active high
      mask Help: Output is active for one-cycle after each edge of the specified type (i.e. rising, falling, or both).  Latency is zero.
      mask TypeOptions edge: Rising | Falling | Both
      mask TypeOptions polarity: Active High | Active Low
      mask Display:
      | plot(x_in_num,0.5+y_in_num*0.2);
      | plot(x_out_num,0.5+y_out_num*0.2);
  edge_detect16 : Subsystem  Commented=on  mask(edge_detect){edge=Rising, polarity=Active High, x_in=[0 0.08 0.08 0.16 0.16 0.24 0.24 0.32 0.32 0.4], y_in=[-1 -1  1  1  1  1  1  1  1  1], x_out=[0.6 0.68 0.68 0.76 0.76 0.84 0.84 0.92 0.92 1], y_out=[-1 -1  1  1 -1 -1 -1 -1 -1 -1]}
      mask prompts: edge "Edge Type"; polarity "Output Polarity"; x_in "Input X Positions"; y_in "Input Y Positions"; x_out "Output X Positions"; y_out "Output Y Positions"
      mask help: Output is active for one-cycle after each edge of the specified type (i.e. rising, falling or both).
      mask init: same as s_c107m32k_vlbi/edge_detect1
      settings: AttributesFormatString=|
      | rising edges
      | active high
      mask Help: Output is active for one-cycle after each edge of the specified type (i.e. rising, falling, or both).  Latency is zero.
      mask TypeOptions edge: Rising | Falling | Both
      mask TypeOptions polarity: Active High | Active Low
      mask Display:
      | plot(x_in_num,0.5+y_in_num*0.2);
      | plot(x_out_num,0.5+y_out_num*0.2);
  edge_detect2 : Subsystem  Commented=on  mask(edge_detect){edge=Rising, polarity=Active High, x_in=[0 0.08 0.08 0.16 0.16 0.24 0.24 0.32 0.32 0.4], y_in=[-1 -1  1  1  1  1  1  1  1  1], x_out=[0.6 0.68 0.68 0.76 0.76 0.84 0.84 0.92 0.92 1], y_out=[-1 -1  1  1 -1 -1 -1 -1 -1 -1]}
      mask prompts: edge "Edge Type"; polarity "Output Polarity"; x_in "Input X Positions"; y_in "Input Y Positions"; x_out "Output X Positions"; y_out "Output Y Positions"
      mask help: Output is active for one-cycle after each edge of the specified type (i.e. rising, falling or both).
      mask init: same as s_c107m32k_vlbi/edge_detect1
      settings: AttributesFormatString=|
      | rising edges
      | active high
      mask Help: Output is active for one-cycle after each edge of the specified type (i.e. rising, falling, or both).  Latency is zero.
      mask TypeOptions edge: Rising | Falling | Both
      mask TypeOptions polarity: Active High | Active Low
      mask Display:
      | plot(x_in_num,0.5+y_in_num*0.2);
      | plot(x_out_num,0.5+y_out_num*0.2);
  edge_detect29 : Subsystem  Commented=on  mask(edge_detect){edge=Rising, polarity=Active High, x_in=[0 0.08 0.08 0.16 0.16 0.24 0.24 0.32 0.32 0.4], y_in=[-1 -1  1  1  1  1  1  1  1  1], x_out=[0.6 0.68 0.68 0.76 0.76 0.84 0.84 0.92 0.92 1], y_out=[-1 -1  1  1 -1 -1 -1 -1 -1 -1]}
      mask prompts: edge "Edge Type"; polarity "Output Polarity"; x_in "Input X Positions"; y_in "Input Y Positions"; x_out "Output X Positions"; y_out "Output Y Positions"
      mask help: Output is active for one-cycle after each edge of the specified type (i.e. rising, falling or both).
      mask init: same as s_c107m32k_vlbi/edge_detect1
      settings: AttributesFormatString=|
      | rising edges
      | active high
      mask Help: Output is active for one-cycle after each edge of the specified type (i.e. rising, falling, or both).  Latency is zero.
      mask TypeOptions edge: Rising | Falling | Both
      mask TypeOptions polarity: Active High | Active Low
      mask Display:
      | plot(x_in_num,0.5+y_in_num*0.2);
      | plot(x_out_num,0.5+y_out_num*0.2);
  edge_detect3 : Subsystem  Commented=on  mask(edge_detect){edge=Falling, polarity=Active High, x_in=[0 0.08 0.08 0.16 0.16 0.24 0.24 0.32 0.32 0.4], y_in=[-1 -1  1  1  1  1  1  1  1  1], x_out=[0.6 0.68 0.68 0.76 0.76 0.84 0.84 0.92 0.92 1], y_out=[-1 -1  1  1 -1 -1 -1 -1 -1 -1]}
      mask prompts: edge "Edge Type"; polarity "Output Polarity"; x_in "Input X Positions"; y_in "Input Y Positions"; x_out "Output X Positions"; y_out "Output Y Positions"
      mask help: Output is active for one-cycle after each edge of the specified type (i.e. rising, falling or both).
      mask init: same as s_c107m32k_vlbi/edge_detect1
      settings: AttributesFormatString=|
      | falling edges
      | active high
      mask Help: Output is active for one-cycle after each edge of the specified type (i.e. rising, falling, or both).  Latency is zero.
      mask TypeOptions edge: Rising | Falling | Both
      mask TypeOptions polarity: Active High | Active Low
      mask Display:
      | plot(x_in_num,0.5+y_in_num*0.2);
      | plot(x_out_num,0.5+y_out_num*0.2);
  edge_detect40 : Subsystem  Commented=on  mask(edge_detect){edge=Rising, polarity=Active High, x_in=[0 0.08 0.08 0.16 0.16 0.24 0.24 0.32 0.32 0.4], y_in=[-1 -1  1  1  1  1  1  1  1  1], x_out=[0.6 0.68 0.68 0.76 0.76 0.84 0.84 0.92 0.92 1], y_out=[-1 -1  1  1 -1 -1 -1 -1 -1 -1]}
      mask prompts: edge "Edge Type"; polarity "Output Polarity"; x_in "Input X Positions"; y_in "Input Y Positions"; x_out "Output X Positions"; y_out "Output Y Positions"
      mask help: Output is active for one-cycle after each edge of the specified type (i.e. rising, falling or both).
      mask init: same as s_c107m32k_vlbi/edge_detect1
      settings: AttributesFormatString=|
      | rising edges
      | active high
      mask Help: Output is active for one-cycle after each edge of the specified type (i.e. rising, falling, or both).  Latency is zero.
      mask TypeOptions edge: Rising | Falling | Both
      mask TypeOptions polarity: Active High | Active Low
      mask Display:
      | plot(x_in_num,0.5+y_in_num*0.2);
      | plot(x_out_num,0.5+y_out_num*0.2);
  edge_detect51 : Subsystem  Commented=on  mask(edge_detect){edge=Falling, polarity=Active High, x_in=[0 0.08 0.08 0.16 0.16 0.24 0.24 0.32 0.32 0.4], y_in=[-1 -1  1  1  1  1  1  1  1  1], x_out=[0.6 0.68 0.68 0.76 0.76 0.84 0.84 0.92 0.92 1], y_out=[-1 -1  1  1 -1 -1 -1 -1 -1 -1]}
      mask prompts: edge "Edge Type"; polarity "Output Polarity"; x_in "Input X Positions"; y_in "Input Y Positions"; x_out "Output X Positions"; y_out "Output Y Positions"
      mask help: Output is active for one-cycle after each edge of the specified type (i.e. rising, falling or both).
      mask init: same as s_c107m32k_vlbi/edge_detect1
      settings: AttributesFormatString=|
      | falling edges
      | active high
      mask Help: Output is active for one-cycle after each edge of the specified type (i.e. rising, falling, or both).  Latency is zero.
      mask TypeOptions edge: Rising | Falling | Both
      mask TypeOptions polarity: Active High | Active Low
      mask Display:
      | plot(x_in_num,0.5+y_in_num*0.2);
      | plot(x_out_num,0.5+y_out_num*0.2);
  pipeline21 : Subsystem  Commented=on  AncestorBlock=casper_library_delays/pipeline  mask(pipeline){latency=2}
      mask help:
      | An explicitly laid-out delay line to avoid mapping to SRL16s
      | for use in pipelining to help achieve timing closure.
      mask init:
      | pipeline_init(gcb,'latency',latency);
      settings: AttributesFormatString=Latency = %<latency>
      mask Display:
      | port_label('input', 1, 'd');
      | port_label('output', 1, 'q');
      | disp(['Z^-', num2str(latency)]);
  pipeline22 : Subsystem  Commented=on  AncestorBlock=casper_library_delays/pipeline  mask(pipeline){latency=2}
      mask help:
      | An explicitly laid-out delay line to avoid mapping to SRL16s
      | for use in pipelining to help achieve timing closure.
      mask init:
      | pipeline_init(gcb,'latency',latency);
      settings: AttributesFormatString=Latency = %<latency>
      mask Display:
      | port_label('input', 1, 'd');
      | port_label('output', 1, 'q');
      | disp(['Z^-', num2str(latency)]);
  pipeline39 : Subsystem  Commented=on  AncestorBlock=casper_library_delays/pipeline  mask(pipeline){latency=2}
      mask help:
      | An explicitly laid-out delay line to avoid mapping to SRL16s
      | for use in pipelining to help achieve timing closure.
      mask init:
      | pipeline_init(gcb,'latency',latency);
      settings: AttributesFormatString=Latency = %<latency>
      mask Display:
      | port_label('input', 1, 'd');
      | port_label('output', 1, 'q');
      | disp(['Z^-', num2str(latency)]);
  pipeline40 : Subsystem  Commented=on  AncestorBlock=casper_library_delays/pipeline  mask(pipeline){latency=2}
      mask help:
      | An explicitly laid-out delay line to avoid mapping to SRL16s
      | for use in pipelining to help achieve timing closure.
      mask init:
      | pipeline_init(gcb,'latency',latency);
      settings: AttributesFormatString=Latency = %<latency>
      mask Display:
      | port_label('input', 1, 'd');
      | port_label('output', 1, 'q');
      | disp(['Z^-', num2str(latency)]);
  ri_to_c1 : casper_library_misc/ri_to_c  Commented=on
      settings: SourceProductName=CASPER DSP Blockset
  sync_lat_decfir : Subsystem  Tag=xps:sw_reg  Commented=on  AncestorBlock=xps_library/Memory/software_register  mask(swreg){io_dir=To Processor, io_delay=0, init_val=0, sample_period=1, names=count, bitwidths=32, bin_pts=0, arith_types=0, sim_port=off, show_format=on}
      mask prompts: io_dir "I/O direction"; io_delay "I/O delay"; init_val "Initial Value"; sample_period "Sample period"; names "Bitfield names [msb...lsb]"; bitwidths "Bitfield widths"; bin_pts "Bitfield binary pts"; arith_types "Bitfield types, ufix=0, fix=1, bool=2"; sim_port "Provide sim input/output?"; show_format "Print format string?"
      mask help: A 32-bit software-accessible register. Can be divided into bitfields of varying widths and types using the fields in the block mask.
      mask init:
      | swreg_init(gcb)
      settings: AttributesFormatString=1output:uf32.0 = 32 bits
      mask TypeOptions io_dir: To Processor | From Processor
      mask Callback io_dir:
      | mask_enables = get_param(gcb, 'MaskEnables');
      | mask_names = get_param(gcb, 'MaskNames');
      | if strcmp(get_param(gcb, 'io_dir'), 'To Processor'),
      |     mask_enables{ismember(mask_names, 'sample_period')} = 'off';
      | else
      |     mask_enables{ismember(mask_names, 'sample_period')} = 'on';
      | end
      | set_param(gcb, 'MaskEnables', mask_enables);
      mask DialogControl ParameterTabVar0 Prompt: Setup
  sync_lat_decfir_free : Subsystem  Tag=xps:sw_reg  Commented=on  AncestorBlock=xps_library/Memory/software_register  mask(swreg){io_dir=To Processor, io_delay=0, init_val=0, sample_period=1, names=count, bitwidths=32, bin_pts=0, arith_types=0, sim_port=off, show_format=on}
      mask prompts: io_dir "I/O direction"; io_delay "I/O delay"; init_val "Initial Value"; sample_period "Sample period"; names "Bitfield names [msb...lsb]"; bitwidths "Bitfield widths"; bin_pts "Bitfield binary pts"; arith_types "Bitfield types, ufix=0, fix=1, bool=2"; sim_port "Provide sim input/output?"; show_format "Print format string?"
      mask help: A 32-bit software-accessible register. Can be divided into bitfields of varying widths and types using the fields in the block mask.
      mask init:
      | swreg_init(gcb)
      settings: AttributesFormatString=1output:uf32.0 = 32 bits
      mask TypeOptions io_dir: To Processor | From Processor
      mask Callback io_dir:
      | mask_enables = get_param(gcb, 'MaskEnables');
      | mask_names = get_param(gcb, 'MaskNames');
      | if strcmp(get_param(gcb, 'io_dir'), 'To Processor'),
      |     mask_enables{ismember(mask_names, 'sample_period')} = 'off';
      | else
      |     mask_enables{ismember(mask_names, 'sample_period')} = 'on';
      | end
      | set_param(gcb, 'MaskEnables', mask_enables);
      mask DialogControl ParameterTabVar0 Prompt: Setup
  sync_lat_mix : Subsystem  Tag=xps:sw_reg  Commented=on  AncestorBlock=xps_library/Memory/software_register  mask(swreg){io_dir=To Processor, io_delay=0, init_val=0, sample_period=1, names=count, bitwidths=32, bin_pts=0, arith_types=0, sim_port=off, show_format=on}
      mask prompts: io_dir "I/O direction"; io_delay "I/O delay"; init_val "Initial Value"; sample_period "Sample period"; names "Bitfield names [msb...lsb]"; bitwidths "Bitfield widths"; bin_pts "Bitfield binary pts"; arith_types "Bitfield types, ufix=0, fix=1, bool=2"; sim_port "Provide sim input/output?"; show_format "Print format string?"
      mask help: A 32-bit software-accessible register. Can be divided into bitfields of varying widths and types using the fields in the block mask.
      mask init:
      | swreg_init(gcb)
      settings: AttributesFormatString=1output:uf32.0 = 32 bits
      mask TypeOptions io_dir: To Processor | From Processor
      mask Callback io_dir:
      | mask_enables = get_param(gcb, 'MaskEnables');
      | mask_names = get_param(gcb, 'MaskNames');
      | if strcmp(get_param(gcb, 'io_dir'), 'To Processor'),
      |     mask_enables{ismember(mask_names, 'sample_period')} = 'off';
      | else
      |     mask_enables{ismember(mask_names, 'sample_period')} = 'on';
      | end
      | set_param(gcb, 'MaskEnables', mask_enables);
      mask DialogControl ParameterTabVar0 Prompt: Setup
  sync_lat_mix_free : Subsystem  Tag=xps:sw_reg  Commented=on  AncestorBlock=xps_library/Memory/software_register  mask(swreg){io_dir=To Processor, io_delay=0, init_val=0, sample_period=1, names=count, bitwidths=32, bin_pts=0, arith_types=0, sim_port=off, show_format=on}
      mask prompts: io_dir "I/O direction"; io_delay "I/O delay"; init_val "Initial Value"; sample_period "Sample period"; names "Bitfield names [msb...lsb]"; bitwidths "Bitfield widths"; bin_pts "Bitfield binary pts"; arith_types "Bitfield types, ufix=0, fix=1, bool=2"; sim_port "Provide sim input/output?"; show_format "Print format string?"
      mask help: A 32-bit software-accessible register. Can be divided into bitfields of varying widths and types using the fields in the block mask.
      mask init:
      | swreg_init(gcb)
      settings: AttributesFormatString=1output:uf32.0 = 32 bits
      mask TypeOptions io_dir: To Processor | From Processor
      mask Callback io_dir:
      | mask_enables = get_param(gcb, 'MaskEnables');
      | mask_names = get_param(gcb, 'MaskNames');
      | if strcmp(get_param(gcb, 'io_dir'), 'To Processor'),
      |     mask_enables{ismember(mask_names, 'sample_period')} = 'off';
      | else
      |     mask_enables{ismember(mask_names, 'sample_period')} = 'on';
      | end
      | set_param(gcb, 'MaskEnables', mask_enables);
      mask DialogControl ParameterTabVar0 Prompt: Setup
  sync_latch_decfir : Subsystem  Tag=xps:sw_reg  Commented=on  AncestorBlock=xps_library/Memory/software_register  mask(swreg){io_dir=To Processor, io_delay=0, init_val=0, sample_period=1, names=count, bitwidths=32, bin_pts=0, arith_types=0, sim_port=off, show_format=on}
      mask prompts: io_dir "I/O direction"; io_delay "I/O delay"; init_val "Initial Value"; sample_period "Sample period"; names "Bitfield names [msb...lsb]"; bitwidths "Bitfield widths"; bin_pts "Bitfield binary pts"; arith_types "Bitfield types, ufix=0, fix=1, bool=2"; sim_port "Provide sim input/output?"; show_format "Print format string?"
      mask help: A 32-bit software-accessible register. Can be divided into bitfields of varying widths and types using the fields in the block mask.
      mask init:
      | swreg_init(gcb)
      settings: AttributesFormatString=1output:uf32.0 = 32 bits
      mask TypeOptions io_dir: To Processor | From Processor
      mask Callback io_dir:
      | mask_enables = get_param(gcb, 'MaskEnables');
      | mask_names = get_param(gcb, 'MaskNames');
      | if strcmp(get_param(gcb, 'io_dir'), 'To Processor'),
      |     mask_enables{ismember(mask_names, 'sample_period')} = 'off';
      | else
      |     mask_enables{ismember(mask_names, 'sample_period')} = 'on';
      | end
      | set_param(gcb, 'MaskEnables', mask_enables);
      mask DialogControl ParameterTabVar0 Prompt: Setup
  sync_latch_mix : Subsystem  Tag=xps:sw_reg  Commented=on  AncestorBlock=xps_library/Memory/software_register  mask(swreg){io_dir=To Processor, io_delay=0, init_val=0, sample_period=1, names=count, bitwidths=32, bin_pts=0, arith_types=0, sim_port=off, show_format=on}
      mask prompts: io_dir "I/O direction"; io_delay "I/O delay"; init_val "Initial Value"; sample_period "Sample period"; names "Bitfield names [msb...lsb]"; bitwidths "Bitfield widths"; bin_pts "Bitfield binary pts"; arith_types "Bitfield types, ufix=0, fix=1, bool=2"; sim_port "Provide sim input/output?"; show_format "Print format string?"
      mask help: A 32-bit software-accessible register. Can be divided into bitfields of varying widths and types using the fields in the block mask.
      mask init:
      | swreg_init(gcb)
      settings: AttributesFormatString=1output:uf32.0 = 32 bits
      mask TypeOptions io_dir: To Processor | From Processor
      mask Callback io_dir:
      | mask_enables = get_param(gcb, 'MaskEnables');
      | mask_names = get_param(gcb, 'MaskNames');
      | if strcmp(get_param(gcb, 'io_dir'), 'To Processor'),
      |     mask_enables{ismember(mask_names, 'sample_period')} = 'off';
      | else
      |     mask_enables{ismember(mask_names, 'sample_period')} = 'on';
      | end
      | set_param(gcb, 'MaskEnables', mask_enables);
      mask DialogControl ParameterTabVar0 Prompt: Setup
  we_delay1 : Subsystem  Tag=cmac_delinked  Commented=on  mask(pipeline){csp_latency=2}
      mask prompts: csp_latency "Latency"
      mask help:
      | An explicitly laid-out delay line to avoid mapping to SRL16s
      | for use in pipelining to help achieve timing closure.
      mask init:
      | pipeline_init(gcb,'latency',csp_latency);
      settings: AttributesFormatString=Latency = %<latency>
      mask Display:
      | port_label('input', 1, 'd');
      | port_label('output', 1, 'q');
      | disp(['Z^-', num2str(csp_latency)]);
  we_delay2 : Subsystem  Tag=cmac_delinked  Commented=on  mask(pipeline){csp_latency=2}
      mask prompts: csp_latency "Latency"
      mask help:
      | An explicitly laid-out delay line to avoid mapping to SRL16s
      | for use in pipelining to help achieve timing closure.
      mask init:
      | pipeline_init(gcb,'latency',csp_latency);
      settings: AttributesFormatString=Latency = %<latency>
      mask Display:
      | port_label('input', 1, 'd');
      | port_label('output', 1, 'q');
      | disp(['Z^-', num2str(csp_latency)]);
  we_delay3 : Subsystem  Tag=cmac_delinked  Commented=on  mask(pipeline){csp_latency=2}
      mask prompts: csp_latency "Latency"
      mask help:
      | An explicitly laid-out delay line to avoid mapping to SRL16s
      | for use in pipelining to help achieve timing closure.
      mask init:
      | pipeline_init(gcb,'latency',csp_latency);
      settings: AttributesFormatString=Latency = %<latency>
      mask Display:
      | port_label('input', 1, 'd');
      | port_label('output', 1, 'q');
      | disp(['Z^-', num2str(csp_latency)]);
  we_delay33 : Subsystem  Tag=cmac_delinked  Commented=on  mask(pipeline){csp_latency=2}
      mask prompts: csp_latency "Latency"
      mask help:
      | An explicitly laid-out delay line to avoid mapping to SRL16s
      | for use in pipelining to help achieve timing closure.
      mask init:
      | pipeline_init(gcb,'latency',csp_latency);
      settings: AttributesFormatString=Latency = %<latency>
      mask Display:
      | port_label('input', 1, 'd');
      | port_label('output', 1, 'q');
      | disp(['Z^-', num2str(csp_latency)]);
  we_delay54 : Subsystem  Tag=cmac_delinked  Commented=on  mask(pipeline){csp_latency=2}
      mask prompts: csp_latency "Latency"
      mask help:
      | An explicitly laid-out delay line to avoid mapping to SRL16s
      | for use in pipelining to help achieve timing closure.
      mask init:
      | pipeline_init(gcb,'latency',csp_latency);
      settings: AttributesFormatString=Latency = %<latency>
      mask Display:
      | port_label('input', 1, 'd');
      | port_label('output', 1, 'q');
      | disp(['Z^-', num2str(csp_latency)]);
  we_delay66 : Subsystem  Tag=cmac_delinked  Commented=on  mask(pipeline){csp_latency=2}
      mask prompts: csp_latency "Latency"
      mask help:
      | An explicitly laid-out delay line to avoid mapping to SRL16s
      | for use in pipelining to help achieve timing closure.
      mask init:
      | pipeline_init(gcb,'latency',csp_latency);
      settings: AttributesFormatString=Latency = %<latency>
      mask Display:
      | port_label('input', 1, 'd');
      | port_label('output', 1, 'q');
      | disp(['Z^-', num2str(csp_latency)]);
  ddc_sync : Outport
  ddc_pol0 : Outport  Port=2
  ddc_pol1 : Outport  Port=3
  ddc_dv : Outport  Port=4
  ddc_of : Outport  Port=5
  mix_of : Outport  Port=6
  tag scope: dec_d80_0=global, dec_d80_1=global, dec_dv=global, dec_sync=global, mix_80_0=global, mix_dvalid=global, mix_sync=global
  wires:
  Concat/1 -> bus_mult/3(misci)
  [ddc_sync] -> ddc_sync/1
  [ddc_pol0] -> ddc_pol0/1
  [ddc_pol1] -> ddc_pol1/1
  pol1_data/1 -> bus_mult1/1(a)
  osc1/1 -> bus_mult1/2(b)
  From20/1 -> pipeline22/1(d)
  Counter1/1 -> ddc_out_sync_cnt/1(out_reg)
  pipeline21/1(q) -> Counter1/2
  pipeline22/1(q) -> Counter1/1
  From34/1 -> edge_detect16/1(in)
  [ddc_dvalid] -> ddc_dv/1
  Delay3/1 -> bus_expand5/1(bus_in)
  bus_expand1/1(msb_out16) -> dec_fir_async/3(real1)
  bus_expand1/2(out15) -> dec_fir_async/4(imag1)
  bus_expand1/3(out14) -> dec_fir_async/5(real2)
  bus_expand1/4(out13) -> dec_fir_async/6(imag2)
  bus_expand1/5(out12) -> dec_fir_async/7(real3)
  bus_expand1/6(out11) -> dec_fir_async/8(imag3)
  bus_expand1/7(out10) -> dec_fir_async/9(real4)
  bus_expand1/8(out9) -> dec_fir_async/10(imag4)
  bus_expand1/9(out8) -> dec_fir_async/11(real5)
  bus_expand1/10(out7) -> dec_fir_async/12(imag5)
  bus_expand1/11(out6) -> dec_fir_async/13(real6)
  bus_expand1/12(out5) -> dec_fir_async/14(imag6)
  bus_expand1/13(out4) -> dec_fir_async/15(real7)
  bus_expand1/14(out3) -> dec_fir_async/16(imag7)
  bus_expand1/15(out2) -> dec_fir_async/17(real8)
  bus_expand1/16(lsb_out1) -> dec_fir_async/18(imag8)
  bus_expand2/1(msb_out16) -> dec_fir_async/19(real9)
  bus_expand2/3(out14) -> dec_fir_async/21(real10)
  bus_expand2/2(out15) -> dec_fir_async/20(imag9)
  bus_expand2/4(out13) -> dec_fir_async/22(imag10)
  bus_expand2/5(out12) -> dec_fir_async/23(real11)
  bus_expand2/7(out10) -> dec_fir_async/25(real12)
  bus_expand2/6(out11) -> dec_fir_async/24(imag11)
  bus_expand2/8(out9) -> dec_fir_async/26(imag12)
  bus_expand2/9(out8) -> dec_fir_async/27(real13)
  bus_expand2/10(out7) -> dec_fir_async/28(imag13)
  bus_expand2/11(out6) -> dec_fir_async/29(real14)
  bus_expand2/12(out5) -> dec_fir_async/30(imag14)
  bus_expand2/14(out3) -> dec_fir_async/32(imag15)
  bus_expand2/13(out4) -> dec_fir_async/31(real15)
  bus_expand2/15(out2) -> dec_fir_async/33(real16)
  bus_expand2/16(lsb_out1) -> dec_fir_async/34(imag16)
  dec_fir_async/2(dout) -> Delay7/1
  From28/1 -> pipeline40/1(d)
  Counter3/1 -> ddc_in_sync_cnt/1(out_reg)
  pipeline39/1(q) -> Counter3/2
  pipeline40/1(q) -> Counter3/1
  From33/1 -> pipeline39/1(d)
  [dec_dv] -> dec_fir_async/2(dv_in)
  [dec_sync] -> dec_fir_async/1(sync_in)
  [ddc_of_pol0] -> Concat1/1
  [ddc_of_pol1] -> Concat1/2
  Concat1/1 -> ddc_of/1
  bus_expand6/16(lsb_out1) -> dec_fir_async2/34(imag16)
  bus_expand6/15(out2) -> dec_fir_async2/33(real16)
  bus_expand6/14(out3) -> dec_fir_async2/32(imag15)
  bus_expand6/13(out4) -> dec_fir_async2/31(real15)
  bus_expand6/12(out5) -> dec_fir_async2/30(imag14)
  bus_expand6/11(out6) -> dec_fir_async2/29(real14)
  bus_expand6/10(out7) -> dec_fir_async2/28(imag13)
  bus_expand6/9(out8) -> dec_fir_async2/27(real13)
  bus_expand6/8(out9) -> dec_fir_async2/26(imag12)
  bus_expand6/7(out10) -> dec_fir_async2/25(real12)
  bus_expand6/6(out11) -> dec_fir_async2/24(imag11)
  bus_expand6/5(out12) -> dec_fir_async2/23(real11)
  bus_expand6/4(out13) -> dec_fir_async2/22(imag10)
  bus_expand6/3(out14) -> dec_fir_async2/21(real10)
  bus_expand6/2(out15) -> dec_fir_async2/20(imag9)
  bus_expand6/1(msb_out16) -> dec_fir_async2/19(real9)
  bus_expand5/16(lsb_out1) -> dec_fir_async2/18(imag8)
  bus_expand5/15(out2) -> dec_fir_async2/17(real8)
  bus_expand5/14(out3) -> dec_fir_async2/16(imag7)
  bus_expand5/13(out4) -> dec_fir_async2/15(real7)
  bus_expand5/12(out5) -> dec_fir_async2/14(imag6)
  bus_expand5/11(out6) -> dec_fir_async2/13(real6)
  bus_expand5/10(out7) -> dec_fir_async2/12(imag5)
  bus_expand5/9(out8) -> dec_fir_async2/11(real5)
  bus_expand5/8(out9) -> dec_fir_async2/10(imag4)
  bus_expand5/7(out10) -> dec_fir_async2/9(real4)
  bus_expand5/6(out11) -> dec_fir_async2/8(imag3)
  bus_expand5/5(out12) -> dec_fir_async2/7(real3)
  bus_expand5/4(out13) -> dec_fir_async2/6(imag2)
  bus_expand5/3(out14) -> dec_fir_async2/5(real2)
  bus_expand5/2(out15) -> dec_fir_async2/4(imag1)
  bus_expand5/1(msb_out16) -> dec_fir_async2/3(real1)
  convert_of1/1(dout) -> ri_to_c1/2
  convert_of/1(dout) -> ri_to_c1/1
  convert_of/2(of) -> Logical/1
  convert_of1/2(of) -> Logical/2
  Register1/1 -> Logical1/1, Inverter/1
  Delay2/1 -> [dec_dv]
  Delay6/1 -> [dec_sync]
  Inverter/1 -> Assert/1
  Assert/1 -> Register1/1
  [mix_sync] -> Register1/2, Register2/3, Register2/1
  Register2/1 -> Logical2/1
  Logical2/1 -> Register2/2, Delay6/1
  Logical1/1 -> Logical2/2, Delay2/1
  [mix_dvalid] -> Register3/2, Register/2, Logical1/2, Register1/3
  dec_fir_async2/4(dv_out) -> Delay1/1
  osc0/1 -> bus_mult/2(b)
  pol0_data/1 -> bus_mult/1(a)
  bus_expand/1(msb_out2) -> Gateway Out1/1, [mix_sync]
  dec_fir_async2/1(sync_out) -> [ddc_sync]
  Gateway Out1/1 -> To Workspace1/1
  Gateway Out2/1 -> To Workspace2/1
  bus_expand/2(lsb_out1) -> Gateway Out2/1, [mix_dvalid]
  Delay4/1 -> [ddc_pol0]
  Delay1/1 -> [ddc_dvalid]
  dec_fir_async2/2(dout) -> Delay4/1
  [dec_sync] -> dec_fir_async2/1(sync_in)
  [dec_dv] -> dec_fir_async2/2(dv_in)
  [dec_d80_0] -> bus_expand6/1(bus_in), Delay3/1
  Register/1 -> [dec_d80_0]
  Register3/1 -> [dec_d80_1]
  [mix_80_0] -> Register/1
  [mix_80_1] -> Register3/1
  [mix_dvalid] -> Delay3/2
  Delay5/1 -> bus_expand1/1(bus_in)
  [dec_d80_1] -> bus_expand2/1(bus_in), Delay5/1
  [mix_dvalid] -> Delay5/2
  edge_detect16/1(out) -> pipeline21/1(d)
  we_delay1/1(q) -> sync_lat_mix/1(out_count)
  edge_detect29/1(out) -> Register37/3
  Register37/1 -> we_delay54/1(d)
  we_delay54/1(q) -> sync_lat_mix_free/1(out_count)
  From6/1 -> edge_detect29/1(in)
  Counter46/1 -> Register37/1
  edge_detect1/1(out) -> Register5/3
  From13/1 -> Register5/2, Counter4/1
  Register5/1 -> we_delay2/1(d)
  we_delay2/1(q) -> sync_lat_decfir_free/1(out_count)
  From17/1 -> edge_detect1/1(in)
  Counter4/1 -> Register5/1
  edge_detect40/1(out) -> Register49/3
  Slice34/1 -> Register49/1
  From19/1 -> Slice34/1
  we_delay66/1(q) -> sync_latch_mix/1(out_count)
  Register49/1 -> we_delay66/1(d)
  From18/1 -> edge_detect40/1(in)
  edge_detect2/1(out) -> Register6/3
  Slice1/1 -> Register6/1
  From23/1 -> Slice1/1
  we_delay3/1(q) -> sync_latch_decfir/1(out_count)
  Register6/1 -> we_delay3/1(d)
  From21/1 -> Register6/2
  From22/1 -> edge_detect2/1(in)
  edge_detect51/1(out) -> Register62/3
  Register24/1 -> edge_detect51/1(in), Logical29/1
  Counter33/1 -> Register62/1
  Logical29/1 -> Counter33/2
  Register62/1 -> we_delay33/1(d)
  From3/1 -> Logical29/2
  From2/1 -> Register62/2, Counter33/1, Register24/1, Register24/3
  From4/1 -> Register24/2
  we_delay33/1(q) -> sync_lat_decfir/1(out_count)
  edge_detect3/1(out) -> Register7/3
  Register4/1 -> edge_detect3/1(in), Logical3/1
  Counter2/1 -> Register7/1
  Logical3/1 -> Counter2/2
  Register7/1 -> we_delay1/1(d)
  dvalid/1 -> Logical3/2, Concat/2
  sync/1 -> Register7/2, Counter2/1, Register4/1, Register4/3, Register49/2, Register37/2, Counter46/1, Concat/1
  From16/1 -> Register4/2
  Delay7/1 -> [ddc_pol1]
  Delay8/1 -> [ddc_of_pol0]
  dec_fir_async2/3(of_out) -> Delay8/1
  dec_fir_async/3(of_out) -> Delay9/1
  Delay9/1 -> [ddc_of_pol1]
  dec_fir_async/1(sync_out) -> Terminator/1
  dec_fir_async/4(dv_out) -> Terminator1/1
  bus_mult/1(a*b) -> bus_convert/1(din)
  bus_mult/2(misco) -> bus_convert/2(misci)
  bus_convert/1(dout) -> [mix_80_0]
  bus_convert/3(misco) -> bus_expand/1(bus_in)
  bus_convert1/1(dout) -> [mix_80_1]
  bus_mult1/1(a*b) -> bus_convert1/1(din)
  Relational/1 -> [mix_of_pol0]
  Constant/1 -> Relational1/2, Relational/2
  bus_convert/2(overflow) -> Relational/1
  bus_convert1/2(overflow) -> Relational1/1
  Relational1/1 -> [mix_of_pol1]
  [mix_of_pol1] -> Concat2/2
  Concat2/1 -> mix_of/1
  [mix_of_pol0] -> Concat2/1
